simulink model "MCS_STD_PMSM_MODEL_2022b"  (R2022b)
settings: Solver=VariableStepAuto  StartTime=0.0  StopTime=2  RelTol=1e-3
libraries: gmp_peripheral_utilities x11, spsSeriesRLCBranchLib x6, gmp_sil_core_pack x1, spsPermanentMagnetSynchronousMachineLib x1, spsControlledVoltageSourceLib x1, spspowerguiLib x1
settings Model: Creator=javnson  LastModifiedBy=javnson
settings OptimizationCC: ReuseModelBlockBuffer=on
settings RTWCC: GPUComputeCapability=5.0

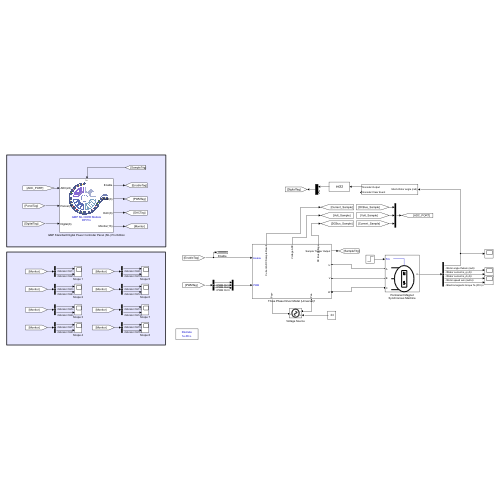
[thumbnail: Simulink's stored preview of the top-level diagram]
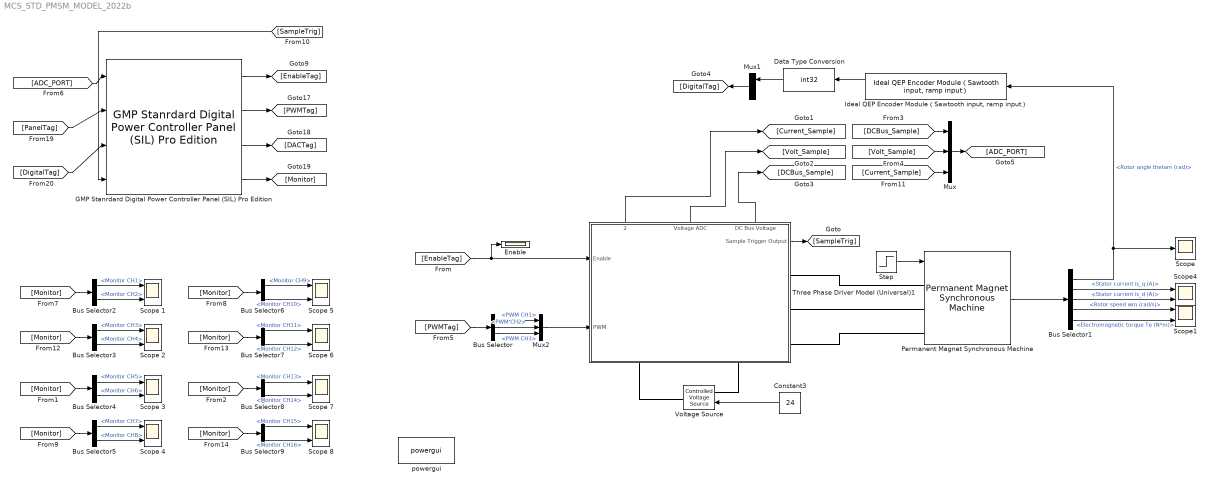
== system MCS_STD_PMSM_MODEL_2022b ==
  Bus Selector : BusSelector  OutputSignals=PWM CH1,PWM CH2,PWM CH3
  Bus Selector1 : BusSelector  OutputSignals=Rotor angle thetam (rad),Stator current is_q (A),Stator current is_d (A),Rotor speed wm (rad/s),Electromagnetic torque Te (N*m)
  Bus Selector2 : BusSelector  OutputSignals=Monitor CH1,Monitor CH2
  Bus Selector3 : BusSelector  OutputSignals=Monitor CH3,Monitor CH4
  Bus Selector4 : BusSelector  OutputSignals=Monitor CH5,Monitor CH6
  Bus Selector5 : BusSelector  OutputSignals=Monitor CH7,Monitor CH8
  Bus Selector6 : BusSelector  OutputSignals=Monitor CH9,Monitor CH10
  Bus Selector7 : BusSelector  OutputSignals=Monitor CH11,Monitor CH12
  Bus Selector8 : BusSelector  OutputSignals=Monitor CH13,Monitor CH14
  Bus Selector9 : BusSelector  OutputSignals=Monitor CH15,Monitor CH16
  Constant3 : Constant  Value=24
  Data Type Conversion : DataTypeConversion  OutDataTypeStr=int32  SaturateOnIntegerOverflow=off  RndMeth=Floor
  Enable : Scope
  GMP Stanrdard Digital Power Controller Panel (SIL) Pro Edition : gmp_sil_core_pack/GMP Stanrdard Digital Power Controller Panel (SIL) Pro Edition
      settings: SourceProductName=GMP SIL Core Utilities
  "Ideal QEP Encoder Module（Sawtooth input, ramp input）" : gmp_peripheral_utilities/Ideal QEP Encoder Module（Sawtooth input, ramp input）  QEP_LINE=4096
      settings: SourceProductName=Virtual Peripheral Utilities
  Mux : Mux  Inputs=3
  Mux1 : Mux  Inputs=2
  Mux2 : Mux  Inputs=3
  Permanent Magnet Synchronous Machine : spsPermanentMagnetSynchronousMachineLib/Permanent Magnet Synchronous Machine  NbPhases=3  FluxDistribution=Sinusoidal  RotorType=Round  MechanicalLoad=Torque Tm  PresetModel=No  ShowDetailedParameters=on  MeasurementBus=off  Resistance=4.7  Inductance=8.5e-3  dqInductances=[8.5e-3,8.5e-3]  La=0.96e-3  MachineConstant=Voltage Constant (V_peak L-L / krpm)  Flux=0.0038197  VoltageCst=1000/206.2  TorqueCst=0.040106  Flat=120  Mechanical=[497e-9 1755e-9 7 0]  PolePairs=4  InitialConditions=[0, 0, 0, 0]  InitialConditions5ph=[0 0 0 0 0 0]  RefAngle=Aligned with phase A axis (original Park)  IterativeDiscreteModel=Trapezoidal non iterative  TsBlock=-1  TsPowergui=0
  Scope : Scope
  Scope {1..8} (8 alike) : Scope  NumInputPorts=2
  Scope1 : Scope  NumInputPorts=2
  Scope4 : Scope  NumInputPorts=2
  Step : Step  After=0.001  SampleTime=0
  Three Phase Driver Model (Universal)1 : Subsystem  mask{fswitch=20e3, CMP_MAX=2500, Deadband_Upper=50, Deadband_Lower=50, Deadband_us=1, phase_shift=0, R_mosfet_on=0.1, Lon=0, Rd=0.01, Vf=0.3, Rs=1e5, Cs=inf, Rsap=0.005, ADC_GAIN=20, ADC_BIT=12, ADC_REFERENCE=3.3, ADC_BIAS=1.65, ADC_INIT=0, VOLTAGE_ADC_GAIN=0.04049127, VOLTAGE_ADC_BIT=12, VOLTAGE_ADC_REFERENCE=3.3, VOLTAGE_ADC_VOLTAGE=0, VOLTAGE_ADC_INIT=0, VOLTAGE_ADC_CUT_FREQ=1143.4, DCBUS_ADC_GAIN=0.04049127, DCBUS_ADC_BIT=12, DCBUS_ADC_REFERENCE=3.3, DCBUS_ADC_BIAS=0, DCBUS_ADC_INIT=0}
      mask init:
      | calculate_deadband(gcb, 'Deadband_Upper', 'Deadband_Lower',	'CMP_MAX', 'fswitch', 'Deadband_us');
      settings: PortSchema="{\"entries\":[{\"content\":{\"sides\":[{\"content\":{\"connectorIds\":[\"In1\",\"In2\"]},\"type\":\"ConnectorPlacement.EquallySpacedRectSide\",\"uuid\":\"3f4c86ad-0582-4f47-8583-a8af9a7f9adc\"},{\"content\":{\"connectorIds\":[\"Out1\",\"RConn1\",\"RConn2\",\"RConn3\"],\"side\":\"RIGHT\"},\"type\":\"ConnectorPlacement.EquallySpacedRectSide\",\"uuid\":\"ae91f325-3014-4188-9063-296f4d5623fa\"},{\"content\":{\"connectorIds\":[\"Out2\",\"Out3\",\"Out4\"],\"side\":\"TOP\"},\"type\":\"ConnectorPlacement.EquallySpacedRectSide\",\"uuid\":\"5f2edb36-6849-4a72-b7bd-4d267f120ce4\"},{\"content\":{\"connectorIds\":[\"RConn4\",\"RConn5\"],\"side\":\"BOTTOM\"},\"type\":\"ConnectorPlacement.EquallySpacedRectSide\",\"uuid\":\"79a111ed-6591-4ced-9242-67ea1247c580\"}]},\"type\":\"ConnectorPlacement.EquallySpacedConnector\",\"uuid\":\"8c66eb8e-d25c-472f-a4a5-d1759225ba1c\"}],\"packageUris\":[\"http://schema.mathworks.com/mf0/Connector/R2020b\"],\"version\":\"1.0\"}"
      mask Callback fswitch: calculate_deadband(gcb, 'Deadband_Upper', 'Deadband_Lower',	'CMP_MAX', 'fswitch', 'Deadband_us');
      mask Callback CMP_MAX: calculate_deadband(gcb, 'Deadband_Upper', 'Deadband_Lower',	'CMP_MAX', 'fswitch', 'Deadband_us');
      mask Callback Deadband_Upper: calculate_deadband(gcb, 'Deadband_Upper', 'Deadband_Lower',	'CMP_MAX', 'fswitch', 'Deadband_us');
      mask Callback Deadband_Lower: calculate_deadband(gcb, 'Deadband_Upper', 'Deadband_Lower',	'CMP_MAX', 'fswitch', 'Deadband_us');
      mask DialogControl DescGroupVar Prompt: Three Phases Bridge Peripheral(3-shunt sample)
      mask DialogControl Control21 Prompt: GMP CTL Simulink Utilities: virtual peripherals
      mask DialogControl DescTextVar Prompt: This module provide a ideal 3-phases bridge peripheral.
      mask DialogControl Container4 Prompt: PWM config
      mask DialogControl ParameterGroupVar Prompt: PWM parameters
      mask DialogControl Control2 Prompt: PWM Frequency (Hz):
      mask DialogControl Control4 Prompt: Full Scale PWM Compare value:
      mask DialogControl Control5 Prompt: Deadband Range Set (CMP Value):
      mask DialogControl Control6 Prompt: Deadband time: DEADBAND_CMP/2/CMP_MAX/fswitch
      mask DialogControl Control22 Prompt: Calculated Deadband, us
      mask DialogControl Control20 Prompt: Initial Phase shift:
      mask DialogControl Container5 Prompt: MOSFET config
      mask DialogControl Container7 Prompt: MOSFET parameters
      mask DialogControl Control7 Prompt: Rds(on), unit Ohm
      mask DialogControl Control8 Prompt: Internal diode inducctance, unit H
      mask DialogControl Control9 Prompt: Internal diode resistance Rd, unit Ohm
      mask DialogControl Control10 Prompt: Internal diode forward voltage Vf, unit V
      mask DialogControl Control11 Prompt: Snubber resistance Rs, unit ohm
      mask DialogControl Control12 Prompt: Snubber Capacitance Cs, unit F
      mask DialogControl Container6 Prompt: 3-shunt Current Sample
      mask DialogControl Control13 Prompt: ADC(p.u.) = (real_voltage * ADC_GAIN + ADC_BIAS)/ADC_REFERENCE
      mask DialogControl Control15 Prompt: Shunt Smaple Res, unit Ohm
      mask DialogControl Control14 Prompt: ADC Voltage Gain (Scale Factor):
      mask DialogControl Control16 Prompt: ADC resolution:
      mask DialogControl Control17 Prompt: ADC reference Voltage(V)
      mask DialogControl Control18 Prompt: ADC Bias Voltage(V)
      mask DialogControl Control19 Prompt: ADC Initial Voltage Output (V):
      mask DialogControl Container9 Prompt: 3-shunt Voltage Sample
      mask DialogControl Control34 Prompt: ADC Voltage Gain (Scale Factor):
      mask DialogControl Control23 Prompt: ADC resolution:
      mask DialogControl Control24 Prompt: ADC reference voltage (V), when VOLTAGE_ADC_GAIN = 1, ADC_REF = ADC Full scale
      mask DialogControl Control25 Prompt: ADC Bias Voltage (V):
      mask DialogControl Control26 Prompt: ADC Initial Voltage Output (V):
      mask DialogControl Control27 Prompt: Voltage Filter cut frequency (Hz):
      mask DialogControl Control28 Prompt: Generally, this value less than switch frequency / 10, greater than motor normal frequency * 3
      mask DialogControl Container10 Prompt: DC Bus Voltage Sample
      mask DialogControl Control32 Prompt: ADC reference voltage (V), when VOLTAGE_ADC_GAIN = 1, ADC_REF = ADC Full scale
      mask DialogControl Control29 Prompt: ADC Voltage Gain (Scale Factor):
      mask DialogControl Control30 Prompt: ADC resolution:
      mask DialogControl Control31 Prompt: ADC Bias Voltage (V):
      mask DialogControl Control33 Prompt: ADC Initial Voltage Output (V):
  Voltage Source : spsControlledVoltageSourceLib/Controlled Voltage Source  Initialize=on  Source_Type=AC  Amplitude=0  Phase=0  Frequency=0  Measurements=None
  powergui : spspowerguiLib/powergui  Priority=1  SimulationMode=Discrete  SampleTime=1e-6  frequency=60  Iterations=50  frequencyindice=0  Pbase=100e6  ErrMax=1e-4  UnitsV=kV  UnitsW=MW  buscounter=0  FunctionMessages=off  echomessages=off  EnableUseOfTLC=off  CurrentSourceSwitches=off  DisableSnubberDevices=off  DisableRonSwitches=off  DisableVfSwitches=off  DisplayEquations=off  AutomaticDiscreteSolvers=off  SolverType=Tustin/Backward Euler (TBE)  Interpol=off  ExternalGateDelay=off  methode=off  Ts=100  x0status=blocks  SPID=on  SwTol=0  HookPort=off  NonlinearTolerance=1e-4  nMaxIteration=100  ContinueOnMaxIteration=off  RestoreLinks=warning  ResistiveCurrentMeasurement=off  Frange=[0:2:500]  Ylog=off  Xlog=on  ShowGrid=off  save=off  variable=ZData  structure=0  ZoomFFT=off  StartTime=0.0  cycles=1  DisplayStyle=1  fundamental=60  FreqAxis=off  MaxFrequency=1000  frequencyindicesteady=1  RmsSteady=1  display=off
  wires:
  [PanelTag] -> GMP Stanrdard Digital Power Controller Panel (SIL) Pro Edition/2
  [SampleTrig] -> GMP Stanrdard Digital Power Controller Panel (SIL) Pro Edition/4
  GMP Stanrdard Digital Power Controller Panel (SIL) Pro Edition/2 -> [PWMTag]
  [ADC_PORT] -> GMP Stanrdard Digital Power Controller Panel (SIL) Pro Edition/1
  GMP Stanrdard Digital Power Controller Panel (SIL) Pro Edition/4 -> [Monitor]
  GMP Stanrdard Digital Power Controller Panel (SIL) Pro Edition/1 -> [EnableTag]
  GMP Stanrdard Digital Power Controller Panel (SIL) Pro Edition/3 -> [DACTag]
  [DigitalTag] -> GMP Stanrdard Digital Power Controller Panel (SIL) Pro Edition/3
  Bus Selector1/2 -> Scope4/1  "<Stator current is_q (A)>"
  Step/1 -> Permanent Magnet Synchronous Machine/1
  Mux2/1 -> Three Phase Driver Model (Universal)1/2(PWM)
  Bus Selector1/5 -> Scope1/2  "<Electromagnetic torque Te (N*m)>"
  Three Phase Driver Model (Universal)1/1(Sample Trigger Output) -> [SampleTrig]
  Bus Selector1/4 -> Scope1/1  "<Rotor speed wm (rad/s)>"
  Permanent Magnet Synchronous Machine/1 -> Bus Selector1/1
  Bus Selector1/3 -> Scope4/2  "<Stator current is_d (A)>"
  Bus Selector1/1 -> "Ideal QEP Encoder Module（Sawtooth input, ramp input）"/1, Scope/1  "<Rotor angle thetam (rad)>"
  [EnableTag] -> Enable/1, Three Phase Driver Model (Universal)1/1(Enable)
  Bus Selector8/2 -> Scope 7/2  "<Monitor CH14>"
  Bus Selector2/2 -> Scope 1/2  "<Monitor CH2>"
  Bus Selector4/2 -> Scope 3/2  "<Monitor CH6>"
  Bus Selector3/1 -> Scope 2/1  "<Monitor CH3>"
  [Monitor] -> Bus Selector4/1
  [Monitor] -> Bus Selector7/1
  Bus Selector2/1 -> Scope 1/1  "<Monitor CH1>"
  Bus Selector5/1 -> Scope 4/1  "<Monitor CH7>"
  [Monitor] -> Bus Selector3/1
  Bus Selector8/1 -> Scope 7/1  "<Monitor CH13>"
  Bus Selector3/2 -> Scope 2/2  "<Monitor CH4>"
  Bus Selector4/1 -> Scope 3/1  "<Monitor CH5>"
  Bus Selector7/1 -> Scope 6/1  "<Monitor CH11>"
  [Monitor] -> Bus Selector5/1
  [Monitor] -> Bus Selector8/1
  [Monitor] -> Bus Selector6/1
  Bus Selector6/1 -> Scope 5/1  "<Monitor CH9>"
  Bus Selector5/2 -> Scope 4/2  "<Monitor CH8>"
  [Monitor] -> Bus Selector2/1
  Bus Selector7/2 -> Scope 6/2  "<Monitor CH12>"
  Bus Selector6/2 -> Scope 5/2  "<Monitor CH10>"
  Bus Selector/1 -> Mux2/1  "<PWM CH1>"
  Bus Selector/3 -> Mux2/3  "<PWM CH3>"
  Bus Selector/2 -> Mux2/2  "<PWM CH2>"
  [PWMTag] -> Bus Selector/1
  Three Phase Driver Model (Universal)1/2(Current ADC Sample Result) -> [Current_Sample]
  Three Phase Driver Model (Universal)1/3(Voltage ADC) -> [Volt_Sample]
  Three Phase Driver Model (Universal)1/4(DC Bus Voltage) -> [DCBus_Sample]
  Mux/1 -> [ADC_PORT]
  [DCBus_Sample] -> Mux/1
  [Volt_Sample] -> Mux/2
  [Current_Sample] -> Mux/3
  Mux1/1 -> [DigitalTag]
  Constant3/1 -> Voltage Source/1
  Bus Selector9/1 -> Scope 8/1  "<Monitor CH15>"
  [Monitor] -> Bus Selector9/1
  Bus Selector9/2 -> Scope 8/2  "<Monitor CH16>"
  Data Type Conversion/1 -> Mux1/1
  "Ideal QEP Encoder Module（Sawtooth input, ramp input）"/1 -> Data Type Conversion/1
  connections:
  Three Phase Driver Model (Universal)1/RConn1 -- Permanent Magnet Synchronous Machine/LConn1
  Three Phase Driver Model (Universal)1/RConn2 -- Permanent Magnet Synchronous Machine/LConn2
  Three Phase Driver Model (Universal)1/RConn3 -- Permanent Magnet Synchronous Machine/LConn3
  Three Phase Driver Model (Universal)1/RConn5 -- Voltage Source/LConn1
  Three Phase Driver Model (Universal)1/RConn4 -- Voltage Source/RConn1

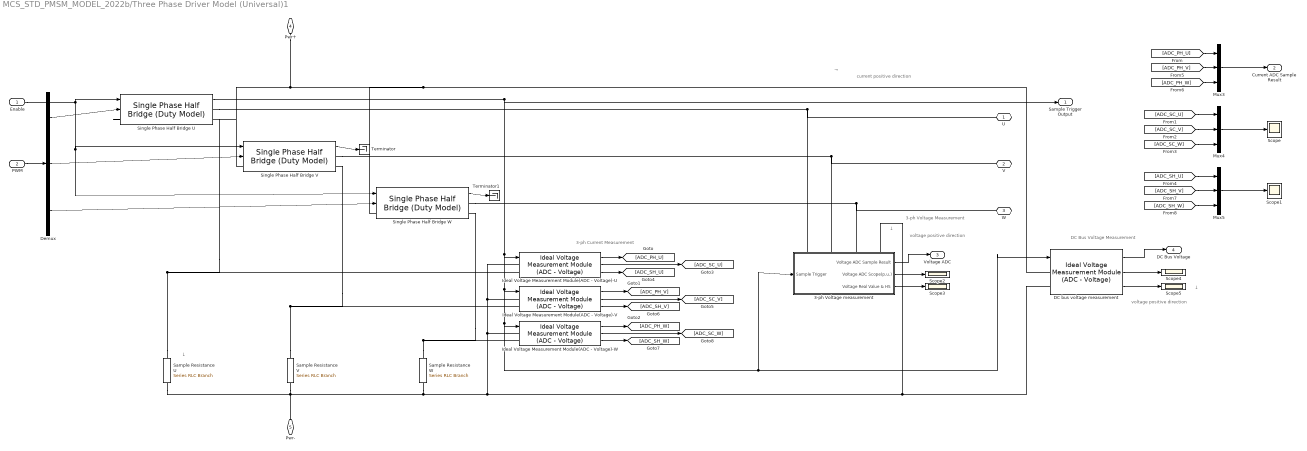
== system MCS_STD_PMSM_MODEL_2022b/Three Phase Driver Model (Universal)1 ==
  note: 3-ph Current Measurement
  note: →
  note: current positive direction
  note: ↓
  note: voltage positive direction
  note: ↓
  note: 3-ph Voltage Measurement
  note: DC Bus Voltage Measurement
  note: ↓
  note: voltage positive direction
  Enable : Inport
  PWM : Inport  Port=2
  3-ph Voltage measurement : Subsystem  mask{ADC_GAIN=VOLTAGE_ADC_GAIN, ADC_BIT=VOLTAGE_ADC_BIT, ADC_REFERENCE=VOLTAGE_ADC_REFERENCE, ADC_BIAS=VOLTAGE_ADC_VOLTAGE, ADC_INIT=VOLTAGE_ADC_INIT, cut_frequency=VOLTAGE_ADC_CUT_FREQ}
      settings: PortSchema="{\"entries\":[{\"content\":{\"sides\":[{\"content\":{\"connectorIds\":[\"In1\"]},\"type\":\"ConnectorPlacement.EquallySpacedRectSide\",\"uuid\":\"ae4f4612-c092-4fa0-8a43-5c9e823110e3\"},{\"content\":{\"connectorIds\":[\"Out1\",\"Out2\",\"Out3\"],\"side\":\"RIGHT\"},\"type\":\"ConnectorPlacement.EquallySpacedRectSide\",\"uuid\":\"6db15ef0-d33a-4775-b4e6-14a566796673\"},{\"content\":{\"connectorIds\":[\"LConn1\",\"LConn2\",\"LConn3\",\"LConn4\"],\"side\":\"TOP\"},\"type\":\"ConnectorPlacement.EquallySpacedRectSide\",\"uuid\":\"cfddd664-59f3-497b-b33e-fe832fe7a7bd\"}]},\"type\":\"ConnectorPlacement.EquallySpacedConnector\",\"uuid\":\"5bacf0ad-0c4a-4f47-a242-d8a476ab7f52\"}],\"packageUris\":[\"http://schema.mathworks.com/mf0/Connector/R2020b\"],\"version\":\"1.0\"}"
      mask DialogControl DescGroupVar Prompt: 3 phases Voltage Sample ADC Model
      mask DialogControl Control10 Prompt: GMP CTL Simulink Utilities: virtual peripherals
      mask DialogControl DescTextVar Prompt: This is a ideal Voltage Measurement Module.
      mask DialogControl Control2 Prompt: ADC(p.u.) = (real_voltage * ADC_GAIN + ADC_BIAS)/ADC_REFERENCE
      mask DialogControl ParameterGroupVar Prompt: parameters:
      mask DialogControl Control3 Prompt: ADC Voltage Gain (Scale Factor):
      mask DialogControl Control4 Prompt: ADC resolution:
      mask DialogControl Control5 Prompt: ADC reference Voltage (V), when ADC_GAIN=1, ADC_REF = ADC full scale
      mask DialogControl Control6 Prompt: ADC Bias Voltage(V)
      mask DialogControl Control7 Prompt: ADC Initial Voltage Output (V):
      mask DialogControl Control8 Prompt: Voltage Filter cut frequency (Hz):
      mask DialogControl Control9 Prompt: Generally, this value less than switch frequency / 10, greater than motor normal frequency * 3
  DC bus voltage measurement : gmp_peripheral_utilities/Ideal Voltage Measurement Module (ADC - Voltage)  ADC_GAIN=DCBUS_ADC_GAIN  ADC_BIT=DCBUS_ADC_BIT  ADC_REFERENCE=DCBUS_ADC_REFERENCE  ADC_BIAS=DCBUS_ADC_BIAS  ADC_INIT=DCBUS_ADC_INIT
      settings: SourceProductName=Virtual Peripheral Utilities
  Demux : Demux  Outputs=3
  Ideal Voltage Measurement Module(ADC - Voltage)-U : gmp_peripheral_utilities/Ideal Voltage Measurement Module (ADC - Voltage)  ADC_GAIN=ADC_GAIN  ADC_BIT=ADC_BIT  ADC_REFERENCE=ADC_REFERENCE  ADC_BIAS=ADC_BIAS  ADC_INIT=ADC_INIT
      settings: SourceProductName=Virtual Peripheral Utilities
  Ideal Voltage Measurement Module(ADC - Voltage)-V : gmp_peripheral_utilities/Ideal Voltage Measurement Module (ADC - Voltage)  ADC_GAIN=ADC_GAIN  ADC_BIT=ADC_BIT  ADC_REFERENCE=ADC_REFERENCE  ADC_BIAS=ADC_BIAS  ADC_INIT=ADC_INIT
      settings: SourceProductName=Virtual Peripheral Utilities
  Ideal Voltage Measurement Module(ADC - Voltage)-W : gmp_peripheral_utilities/Ideal Voltage Measurement Module (ADC - Voltage)  ADC_GAIN=ADC_GAIN  ADC_BIT=ADC_BIT  ADC_REFERENCE=ADC_REFERENCE  ADC_BIAS=ADC_BIAS  ADC_INIT=ADC_INIT
      settings: SourceProductName=Virtual Peripheral Utilities
  Mux3 : Mux  Inputs=3
  Mux4 : Mux  Inputs=3
  Mux5 : Mux  Inputs=3
  Sample Resistance U : spsSeriesRLCBranchLib/Series RLC Branch  LConnTagsString=__new0  RConnTagsString=__new0  BranchType=R  Resistance=Rsap  Inductance=1e-3  SetiL0=off  InitialCurrent=0  Capacitance=1e-6  Setx0=off  InitialVoltage=0  Measurements=None
  Sample Resistance V : spsSeriesRLCBranchLib/Series RLC Branch  LConnTagsString=__new0  RConnTagsString=__new0  BranchType=R  Resistance=Rsap  Inductance=1e-3  SetiL0=off  InitialCurrent=0  Capacitance=1e-6  Setx0=off  InitialVoltage=0  Measurements=None
  Sample Resistance W : spsSeriesRLCBranchLib/Series RLC Branch  LConnTagsString=__new0  RConnTagsString=__new0  BranchType=R  Resistance=Rsap  Inductance=1e-3  SetiL0=off  InitialCurrent=0  Capacitance=1e-6  Setx0=off  InitialVoltage=0  Measurements=None
  Scope{,1..5} (6 alike) : Scope
  Single Phase Half Bridge U : gmp_peripheral_utilities/Single Phase Half Bridge (Duty Model)  fswitch=fswitch  CMP_MAX=CMP_MAX  Deadband_Upper=Deadband_Upper  Deadband_Lower=Deadband_Lower  Deadband_us=NaN  phase_shift=phase_shift  R_mosfet_on=R_mosfet_on  Lon=Lon  Rd=Rd  Vf=Vf  Rs=Rs  Cs=Cs
      settings: SourceProductName=Virtual Peripheral Utilities
  Single Phase Half Bridge V : gmp_peripheral_utilities/Single Phase Half Bridge (Duty Model)  fswitch=fswitch  CMP_MAX=CMP_MAX  Deadband_Upper=Deadband_Upper  Deadband_Lower=Deadband_Lower  Deadband_us=NaN  phase_shift=phase_shift  R_mosfet_on=R_mosfet_on  Lon=Lon  Rd=Rd  Vf=Vf  Rs=Rs  Cs=Cs
      settings: SourceProductName=Virtual Peripheral Utilities
  Single Phase Half Bridge W : gmp_peripheral_utilities/Single Phase Half Bridge (Duty Model)  fswitch=fswitch  CMP_MAX=CMP_MAX  Deadband_Upper=Deadband_Upper  Deadband_Lower=Deadband_Lower  Deadband_us=NaN  phase_shift=phase_shift  R_mosfet_on=R_mosfet_on  Lon=Lon  Rd=Rd  Vf=Vf  Rs=Rs  Cs=Cs
      settings: SourceProductName=Virtual Peripheral Utilities
  Terminator : Terminator
  Terminator1 : Terminator
  U : PMIOPort  Side=Right
  V : PMIOPort  Port=2  Side=Right
  W : PMIOPort  Port=3  Side=Right
  Pwr+ : PMIOPort  Port=4  Side=Right
  Pwr- : PMIOPort  Port=5  Side=Right
  Sample Trigger Output : Outport
  Current ADC Sample Result : Outport  Port=2
  Voltage ADC : Outport  Port=3
  DC Bus Voltage : Outport  Port=4
  wires:
  Ideal Voltage Measurement Module(ADC - Voltage)-U/1 -> [ADC_PH_U]
  Single Phase Half Bridge V/1 -> Terminator/1
  Single Phase Half Bridge W/1 -> Terminator1/1
  Ideal Voltage Measurement Module(ADC - Voltage)-U/2 -> [ADC_SC_U]
  [ADC_PH_V] -> Mux3/2
  [ADC_SC_V] -> Mux4/2
  Ideal Voltage Measurement Module(ADC - Voltage)-U/3 -> [ADC_SH_U]
  Mux3/1 -> Current ADC Sample Result/1
  Ideal Voltage Measurement Module(ADC - Voltage)-V/1 -> [ADC_PH_V]
  [ADC_SC_U] -> Mux4/1
  [ADC_SH_W] -> Mux5/3
  Mux5/1 -> Scope1/1
  Ideal Voltage Measurement Module(ADC - Voltage)-W/1 -> [ADC_PH_W]
  [ADC_PH_U] -> Mux3/1
  Enable/1 -> Single Phase Half Bridge W/1, Single Phase Half Bridge V/1, Single Phase Half Bridge U/1
  Mux4/1 -> Scope/1
  Ideal Voltage Measurement Module(ADC - Voltage)-V/3 -> [ADC_SH_V]
  Single Phase Half Bridge U/1 -> Ideal Voltage Measurement Module(ADC - Voltage)-V/1, Ideal Voltage Measurement Module(ADC - Voltage)-W/1, DC bus voltage measurement/1, 3-ph Voltage measurement/1(Sample Trigger), Ideal Voltage Measurement Module(ADC - Voltage)-U/1, Sample Trigger Output/1
  [ADC_SH_U] -> Mux5/1
  Ideal Voltage Measurement Module(ADC - Voltage)-V/2 -> [ADC_SC_V]
  Ideal Voltage Measurement Module(ADC - Voltage)-W/3 -> [ADC_SH_W]
  [ADC_PH_W] -> Mux3/3
  [ADC_SC_W] -> Mux4/3
  [ADC_SH_V] -> Mux5/2
  Ideal Voltage Measurement Module(ADC - Voltage)-W/2 -> [ADC_SC_W]
  3-ph Voltage measurement/1(Voltage ADC Sample Result) -> Voltage ADC/1
  3-ph Voltage measurement/2(Voltage ADC Scope(p.u.)) -> Scope2/1
  3-ph Voltage measurement/3(Voltage Real Value & HS) -> Scope3/1
  DC bus voltage measurement/1 -> DC Bus Voltage/1
  DC bus voltage measurement/2 -> Scope4/1
  DC bus voltage measurement/3 -> Scope5/1
  Demux/2 -> Single Phase Half Bridge V/2
  Demux/1 -> Single Phase Half Bridge U/2
  Demux/3 -> Single Phase Half Bridge W/2
  PWM/1 -> Demux/1
  connections:
  Single Phase Half Bridge V/RConn1 -- 3-ph Voltage measurement/LConn2 -- V/RConn1
  Single Phase Half Bridge U/RConn1 -- U/RConn1 -- 3-ph Voltage measurement/LConn1
  Single Phase Half Bridge W/RConn1 -- W/RConn1 -- 3-ph Voltage measurement/LConn3
  Sample Resistance V/LConn1 -- Ideal Voltage Measurement Module(ADC - Voltage)-V/LConn2 -- Single Phase Half Bridge V/RConn2
  Pwr-/RConn1 -- Sample Resistance U/RConn1 -- Sample Resistance V/RConn1 -- Sample Resistance W/RConn1 -- 3-ph Voltage measurement/LConn4 -- DC bus voltage measurement/LConn2 -- Ideal Voltage Measurement Module(ADC - Voltage)-U/LConn1 -- Ideal Voltage Measurement Module(ADC - Voltage)-V/LConn1 -- Ideal Voltage Measurement Module(ADC - Voltage)-W/LConn1
  Sample Resistance W/LConn1 -- Ideal Voltage Measurement Module(ADC - Voltage)-W/LConn2 -- Single Phase Half Bridge W/RConn2
  Sample Resistance U/LConn1 -- Ideal Voltage Measurement Module(ADC - Voltage)-U/LConn2 -- Single Phase Half Bridge U/RConn2
  Pwr+/RConn1 -- Single Phase Half Bridge W/LConn1 -- DC bus voltage measurement/LConn1 -- Single Phase Half Bridge U/LConn1 -- Single Phase Half Bridge V/LConn1

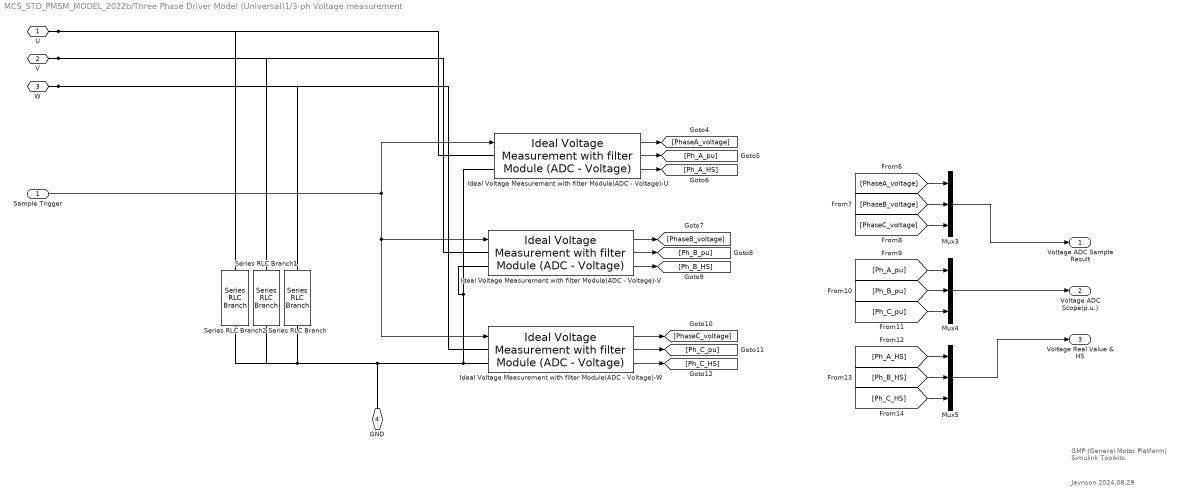
== system MCS_STD_PMSM_MODEL_2022b/Three Phase Driver Model (Universal)1/3-ph Voltage measurement ==
  note: Javnson
      | 2024.08.29
  note: GMP (General Motor Platform)
      | Simulink Toolkits
  Sample Trigger : Inport
  Ideal Voltage Measurement with filter Module(ADC - Voltage)-U : gmp_peripheral_utilities/Ideal Voltage Measurement with filter Module (ADC - Voltage)  ADC_GAIN=ADC_GAIN  ADC_BIT=ADC_BIT  ADC_REFERENCE=ADC_REFERENCE  ADC_BIAS=ADC_BIAS  ADC_INIT=ADC_INIT  cut_frequency=cut_frequency
      settings: SourceProductName=Virtual Peripheral Utilities
  Ideal Voltage Measurement with filter Module(ADC - Voltage)-V : gmp_peripheral_utilities/Ideal Voltage Measurement with filter Module (ADC - Voltage)  ADC_GAIN=ADC_GAIN  ADC_BIT=ADC_BIT  ADC_REFERENCE=ADC_REFERENCE  ADC_BIAS=ADC_BIAS  ADC_INIT=ADC_INIT  cut_frequency=cut_frequency
      settings: SourceProductName=Virtual Peripheral Utilities
  Ideal Voltage Measurement with filter Module(ADC - Voltage)-W : gmp_peripheral_utilities/Ideal Voltage Measurement with filter Module (ADC - Voltage)  ADC_GAIN=ADC_GAIN  ADC_BIT=ADC_BIT  ADC_REFERENCE=ADC_REFERENCE  ADC_BIAS=ADC_BIAS  ADC_INIT=ADC_INIT  cut_frequency=cut_frequency
      settings: SourceProductName=Virtual Peripheral Utilities
  Mux3 : Mux  Inputs=3
  Mux4 : Mux  Inputs=3
  Mux5 : Mux  Inputs=3
  Series RLC Branch : spsSeriesRLCBranchLib/Series RLC Branch  LConnTagsString=__new0  RConnTagsString=__new0  BranchType=R  Resistance=1e6  Inductance=1e-3  SetiL0=off  InitialCurrent=0  Capacitance=1e-6  Setx0=off  InitialVoltage=0  Measurements=None
  Series RLC Branch1 : spsSeriesRLCBranchLib/Series RLC Branch  LConnTagsString=__new0  RConnTagsString=__new0  BranchType=R  Resistance=1e6  Inductance=1e-3  SetiL0=off  InitialCurrent=0  Capacitance=1e-6  Setx0=off  InitialVoltage=0  Measurements=None
  Series RLC Branch2 : spsSeriesRLCBranchLib/Series RLC Branch  LConnTagsString=__new0  RConnTagsString=__new0  BranchType=R  Resistance=1e6  Inductance=1e-3  SetiL0=off  InitialCurrent=0  Capacitance=1e-6  Setx0=off  InitialVoltage=0  Measurements=None
  U : PMIOPort  Side=Left
  V : PMIOPort  Port=2  Side=Left
  W : PMIOPort  Port=3  Side=Left
  GND : PMIOPort  Port=4  Side=Left
  Voltage ADC Sample Result : Outport
  Voltage ADC Scope(p.u.) : Outport  Port=2
  Voltage Real Value & HS : Outport  Port=3
  wires:
  Ideal Voltage Measurement with filter Module(ADC - Voltage)-W/3 -> [Ph_C_HS]
  Sample Trigger/1 -> Ideal Voltage Measurement with filter Module(ADC - Voltage)-U/1, Ideal Voltage Measurement with filter Module(ADC - Voltage)-W/1, Ideal Voltage Measurement with filter Module(ADC - Voltage)-V/1
  Ideal Voltage Measurement with filter Module(ADC - Voltage)-V/2 -> [Ph_B_pu]
  Ideal Voltage Measurement with filter Module(ADC - Voltage)-V/3 -> [Ph_B_HS]
  Mux4/1 -> Voltage ADC Scope(p.u.)/1
  [Ph_B_HS] -> Mux5/2
  Ideal Voltage Measurement with filter Module(ADC - Voltage)-W/1 -> [PhaseC_voltage]
  Ideal Voltage Measurement with filter Module(ADC - Voltage)-V/1 -> [PhaseB_voltage]
  Ideal Voltage Measurement with filter Module(ADC - Voltage)-U/1 -> [PhaseA_voltage]
  Ideal Voltage Measurement with filter Module(ADC - Voltage)-U/2 -> [Ph_A_pu]
  [Ph_B_pu] -> Mux4/2
  [PhaseB_voltage] -> Mux3/2
  Ideal Voltage Measurement with filter Module(ADC - Voltage)-U/3 -> [Ph_A_HS]
  Ideal Voltage Measurement with filter Module(ADC - Voltage)-W/2 -> [Ph_C_pu]
  [Ph_A_pu] -> Mux4/1
  [PhaseC_voltage] -> Mux3/3
  [PhaseA_voltage] -> Mux3/1
  [Ph_C_pu] -> Mux4/3
  [Ph_C_HS] -> Mux5/3
  Mux3/1 -> Voltage ADC Sample Result/1
  [Ph_A_HS] -> Mux5/1
  Mux5/1 -> Voltage Real Value & HS/1
  connections:
  Ideal Voltage Measurement with filter Module(ADC - Voltage)-V/LConn2 -- Ideal Voltage Measurement with filter Module(ADC - Voltage)-U/LConn2 -- Series RLC Branch2/RConn1 -- Series RLC Branch1/RConn1 -- Series RLC Branch/RConn1 -- GND/RConn1 -- Ideal Voltage Measurement with filter Module(ADC - Voltage)-W/LConn2
  U/RConn1 -- Series RLC Branch2/LConn1 -- Ideal Voltage Measurement with filter Module(ADC - Voltage)-U/LConn1
  V/RConn1 -- Series RLC Branch1/LConn1 -- Ideal Voltage Measurement with filter Module(ADC - Voltage)-V/LConn1
  W/RConn1 -- Series RLC Branch/LConn1 -- Ideal Voltage Measurement with filter Module(ADC - Voltage)-W/LConn1
